simulink model "loop_adder_a"  (R2026b)
settings: Solver=FixedStepDiscrete  FixedStep=0.1
settings Model: Creator=Fasih  LastModifiedBy=Fasih

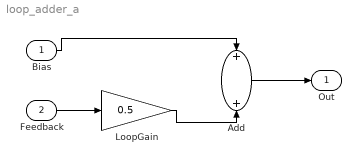
== system loop_adder_a ==
  Bias : Inport
  Feedback : Inport  Port=2
  Add : Sum
  LoopGain : Gain  Gain=0.5
  Out : Outport
  wires:
  Bias/1 -> Add/1
  Feedback/1 -> LoopGain/1
  LoopGain/1 -> Add/2
  Add/1 -> Out/1
